simulink model "mat_model_1_teleso"  (R2025b)
settings: Solver=ode45  StartTime=0.0  StopTime=1800  MaxStep=1  RelTol=1e-3
values from neighbouring files (symbols this model uses):
  A = 7e-4    (= 0.0007)    [u_2_d_1_teleso.m]    (also in u_2_f_1_teleso.m)
  alfa = 0.01    [u_2_d_1_teleso.m]    (also in u_2_f_1_teleso.m)
  c_p = 500    [u_2_d_1_teleso.m]    (also in u_2_f_1_teleso.m)
  epsilon = 0.5    [u_2_d_1_teleso.m]    (also in u_2_f_1_teleso.m)
  m = 0.004    [u_2_d_1_teleso.m]    (also in u_2_f_1_teleso.m)
  sigma = 5.670374e-8    (= 5.670374e-08)    [u_2_d_1_teleso.m]    (also in u_2_f_1_teleso.m)
  T_ok = 23 + 273.15    (= 296.15)    [u_2_d_1_teleso.m]    (also in u_2_f_1_teleso.m = 294.15)
  T_poc = 23 + 273.15    (= 296.15)    [u_2_d_1_teleso.m]    (also in u_2_f_1_teleso.m = 294.15)
  U = 10    [u_2_d_1_teleso.m]    (also in u_2_f_1_teleso.m)
settings Model: Creator=marob  LastModifiedBy=lukas
settings OptimizationCC: BlockReduction=off  DefaultParameterBehavior=Inlined  BufferReuse=off

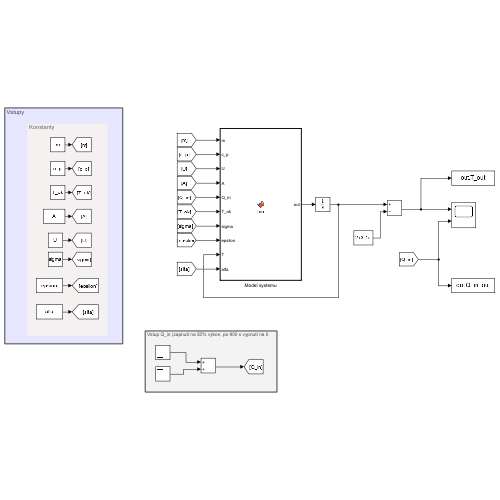
[thumbnail: Simulink's stored preview of the top-level diagram]
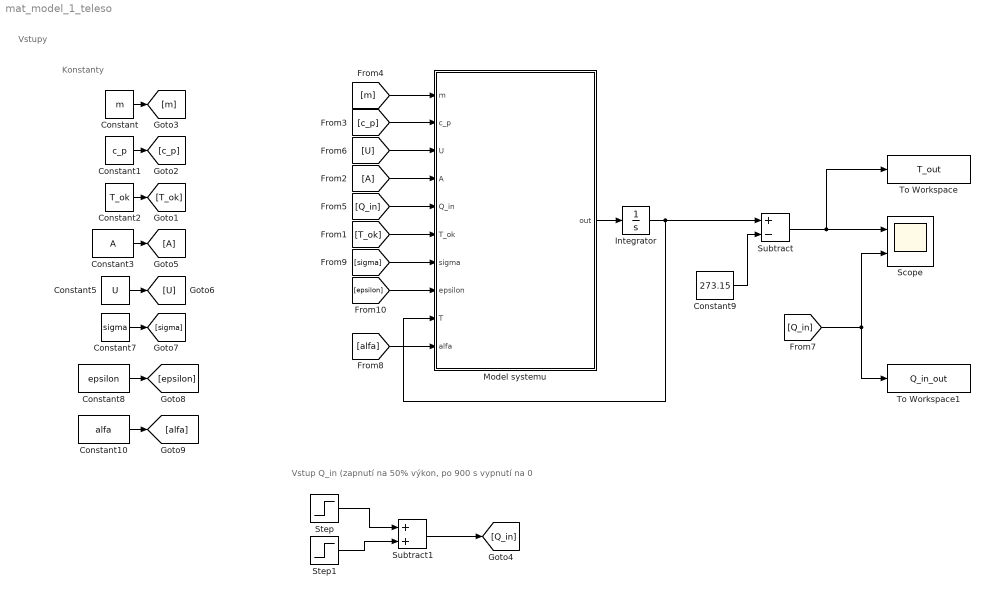
== system mat_model_1_teleso ==
  note: Vstup Q_in (zapnutí na 50% výkon, po 900 s vypnutí na 0
  note: Vstupy
  note: Konstanty
  Constant : Constant  Value=m
  Constant1 : Constant  Value=c_p
  Constant10 : Constant  Value=alfa
  Constant2 : Constant  Value=T_ok
  Constant3 : Constant  Value=A
  Constant5 : Constant  Value=U
  Constant7 : Constant  Value=sigma
  Constant8 : Constant  Value=epsilon
  Constant9 : Constant  Value=273.15
  From2 : From
  Goto5 : Goto
  Integrator : Integrator  InitialCondition=T_poc
  Model systemu : MATLAB Function  TreatAsAtomicUnit=on
  Scope : Scope  NumInputPorts=2
      settings: ActiveDisplayYMinimum=-5.7807366194750989  ActiveDisplayYMaximum=52.0266295752759
  Step : Step  After=50  SampleTime=0
  Step1 : Step  Time=900  After=-50  SampleTime=0
  Subtract : Sum  Inputs=+-
  Subtract1 : Sum
  To Workspace : ToWorkspace  VariableName=T_out  SaveFormat=Timeseries  SampleTime=-1
  To Workspace1 : ToWorkspace  VariableName=Q_in_out  SaveFormat=Timeseries  SampleTime=-1
  wires:
  Model systemu/1(out) -> Integrator/1
  Constant2/1 -> [T_ok]
  Constant/1 -> [m]
  Constant1/1 -> [c_p]
  [c_p] -> Model systemu/2(c_p)
  [m] -> Model systemu/1(m)
  Integrator/1 -> Subtract/1, Model systemu/9(T)
  [Q_in] -> Model systemu/5(Q_in)
  [T_ok] -> Model systemu/6(T_ok)
  Constant3/1 -> Goto5/1
  Constant5/1 -> [U]
  [U] -> Model systemu/3(U)
  From2/1 -> Model systemu/4(A)
  [Q_in] -> To Workspace1/1, Scope/2
  Subtract/1 -> To Workspace/1, Scope/1
  Constant9/1 -> Subtract/2
  Constant7/1 -> [sigma]
  [sigma] -> Model systemu/7(sigma)
  Constant8/1 -> [epsilon]
  [epsilon] -> Model systemu/8(epsilon)
  Constant10/1 -> [alfa]
  [alfa] -> Model systemu/10(alfa)
  Subtract1/1 -> [Q_in]
  Step/1 -> Subtract1/1
  Step1/1 -> Subtract1/2

== matlab function mat_model_1_teleso/Model systemu ==
  data: m input; out output; c_p input; U input; A input; Q_in input; T_ok input; sigma input; epsilon input; T input; alfa input
function out = fcn(m,c_p,U,A,Q_in,T_ok,sigma,epsilon,T, alfa)

out = (1/(m*c_p)) * (alfa*Q_in - U*A*(T-T_ok) - sigma*epsilon*A*( (T^4) - (T_ok^4) ) );
